simulink library "full_bridge_three_level_ttype_ideal_switch_based_model"  (R2025b)
settings: Solver=VariableStepAuto  StartTime=0.0  StopTime=10.0  RelTol=1e-3
libraries: nesl_utility x10, $bdroot x7, fl_lib x5
settings Model: Creator=dbagn  LastModifiedBy=dbagn

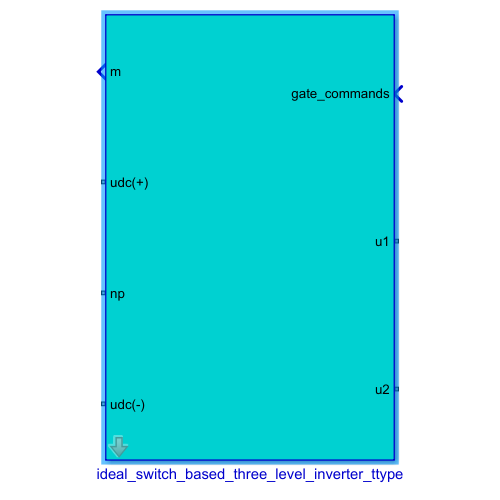
[thumbnail: Simulink's stored preview of the top-level diagram]
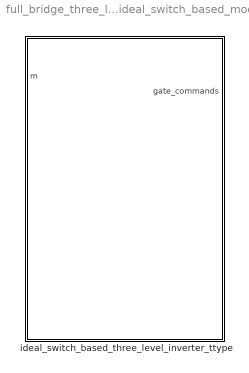
== system full_bridge_three_level_ttype_ideal_switch_based_model ==
  ideal_switch_based_three_level_inverter_ttype : Subsystem  mask{Vth=5.5, Ron=1.5e-3, Vdon_diode=2, Rdon_diode=0.15e-3, Csnubber=10e-9, Rsnubber=2200}

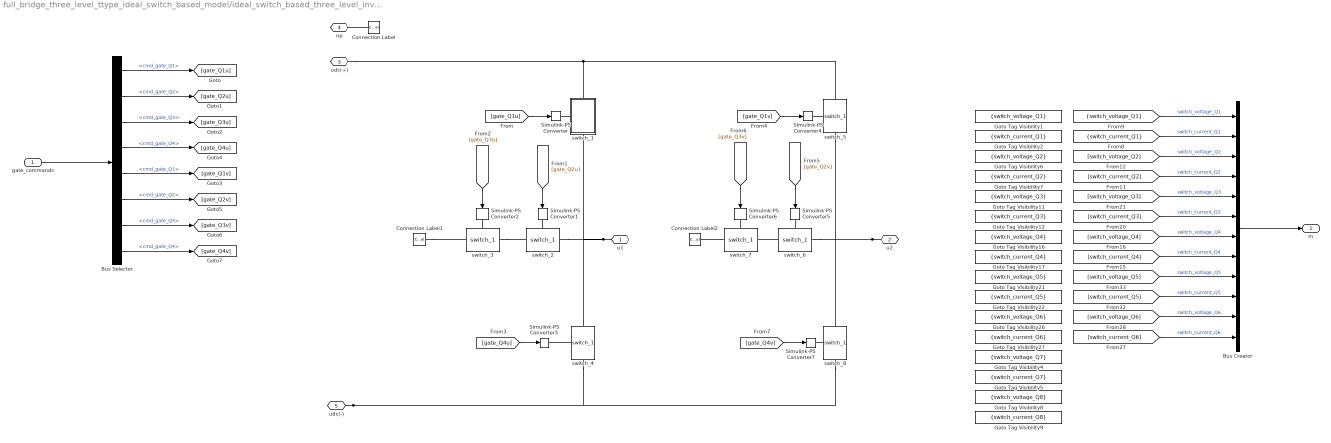
== system full_bridge_three_level_ttype_ideal_switch_based_model/ideal_switch_based_three_level_inverter_ttype ==
  gate_commands : Inport
  Bus Creator : BusCreator  Inputs=12
  Bus Selector : BusSelector  OutputSignals=gate_cmds_ph1.cmd_gate_Q1,gate_cmds_ph1.cmd_gate_Q2,gate_cmds_ph1.cmd_gate_Q3,gate_cmds_ph1.cmd_gate_Q4,gate_cmds_ph2.cmd_gate_Q1,gate_cmds_ph2.cmd_gate_Q2,gate_cmds_ph2.cmd_gate_Q3,gate_cmds_ph2.cmd_gate_Q4
  Connection Label : ConnectionLabel  Label=np
  Connection Label1 : ConnectionLabel  Label=np
  Connection Label2 : ConnectionLabel  Label=np
  Goto Tag Visibility1 : GotoTagVisibility  GotoTag=switch_voltage_Q1
  Goto Tag Visibility11 : GotoTagVisibility  GotoTag=switch_voltage_Q3
  Goto Tag Visibility12 : GotoTagVisibility  GotoTag=switch_current_Q3
  Goto Tag Visibility16 : GotoTagVisibility  GotoTag=switch_voltage_Q4
  Goto Tag Visibility17 : GotoTagVisibility  GotoTag=switch_current_Q4
  Goto Tag Visibility2 : GotoTagVisibility  GotoTag=switch_current_Q1
  Goto Tag Visibility21 : GotoTagVisibility  GotoTag=switch_voltage_Q5
  Goto Tag Visibility22 : GotoTagVisibility  GotoTag=switch_current_Q5
  Goto Tag Visibility26 : GotoTagVisibility  GotoTag=switch_voltage_Q6
  Goto Tag Visibility27 : GotoTagVisibility  GotoTag=switch_current_Q6
  Goto Tag Visibility4 : GotoTagVisibility  GotoTag=switch_voltage_Q7
  Goto Tag Visibility5 : GotoTagVisibility  GotoTag=switch_current_Q7
  Goto Tag Visibility6 : GotoTagVisibility  GotoTag=switch_voltage_Q2
  Goto Tag Visibility7 : GotoTagVisibility  GotoTag=switch_current_Q2
  Goto Tag Visibility8 : GotoTagVisibility  GotoTag=switch_voltage_Q8
  Goto Tag Visibility9 : GotoTagVisibility  GotoTag=switch_current_Q8
  Simulink-PS Converter{,1..7} (8 alike) : nesl_utility/Simulink-PS Converter  PhysicalDomain=network_engine_domain  SubClassName=ps_input  LeftPortType=input  RightPortType=output  PseudoPeriodic=off  Frequencies=[]  NoiseDistribution=none  NoiseParameters=[]  Unit=1  AffineConversion=on  FilteringAndDerivatives=provide  SimscapeFilterOrder=1  InputFilterTimeConstant=0.001  UdotUserProvided=0
  switch_1 : Subsystem
      settings: PortSchema="{\"entries\":[{\"content\":{\"sides\":[{\"content\":{\"connectorIds\":[\"LConn1\"]},\"type\":\"ConnectorPlacement.EquallySpacedRectSide\",\"uuid\":\"9277da8d-d460-43e6-8478-dd662f15d226\"},{\"content\":{\"connectorIds\":[],\"side\":\"RIGHT\"},\"type\":\"ConnectorPlacement.EquallySpacedRectSide\",\"uuid\":\"a7ece396-f1d9-4f4f-a05b-db1fc65d6e1d\"},{\"content\":{\"connectorIds\":[\"LConn2\"],\"side\":\"TOP\"},\"type\":\"ConnectorPlacement.EquallySpacedRectSide\",\"uuid\":\"fdd70777-e9cf-4317-afb6-cae87f75d5b0\"},{\"content\":{\"connectorIds\":[\"RConn1\"],\"side\":\"BOTTOM\"},\"type\":\"ConnectorPlacement.EquallySpacedRectSide\",\"uuid\":\"2353ed68-b1a1-4775-9ca9-31e268d5443b\"}]},\"type\":\"ConnectorPlacement.EquallySpacedConnector\",\"uuid\":\"d5479f4c-4e65-4791-adcb-73df11f88590\"}],\"packageUris\":[\"http://schema.mathworks.com/mf0/Connector/R2020b\"],\"version\":\"1.0\"}"
  switch_2 : $bdroot/ideal_switch_based_three_level_inverter_ttype/switch_1  SystemSampleTime=-1  VariantActivationTime=update diagram  EmptyChoice=off  PassThrough=off  PassThroughVariantControl=(default)  EmptyChoiceVariantControl=(default)  AllowFlexibleInterface=on  Latency=0  AutoFrameSizeCalculation=off
      link override Goto3: GotoTag=switch_voltage_Q2
      link override Goto6: GotoTag=switch_current_Q2
      settings: PortSchema="{\"entries\":[{\"content\":{\"sides\":[{\"content\":{\"connectorIds\":[\"LConn1\"]},\"type\":\"ConnectorPlacement.EquallySpacedRectSide\",\"uuid\":\"9277da8d-d460-43e6-8478-dd662f15d226\"},{\"content\":{\"connectorIds\":[],\"side\":\"RIGHT\"},\"type\":\"ConnectorPlacement.EquallySpacedRectSide\",\"uuid\":\"a7ece396-f1d9-4f4f-a05b-db1fc65d6e1d\"},{\"content\":{\"connectorIds\":[\"LConn2\"],\"side\":\"TOP\"},\"type\":\"ConnectorPlacement.EquallySpacedRectSide\",\"uuid\":\"fdd70777-e9cf-4317-afb6-cae87f75d5b0\"},{\"content\":{\"connectorIds\":[\"RConn1\"],\"side\":\"BOTTOM\"},\"type\":\"ConnectorPlacement.EquallySpacedRectSide\",\"uuid\":\"2353ed68-b1a1-4775-9ca9-31e268d5443b\"}]},\"type\":\"ConnectorPlacement.EquallySpacedConnector\",\"uuid\":\"d5479f4c-4e65-4791-adcb-73df11f88590\"}],\"packageUris\":[\"http://schema.mathworks.com/mf0/Connector/R2020b\"],\"version\":\"1.0\"}"
  switch_3 : $bdroot/ideal_switch_based_three_level_inverter_ttype/switch_1  SystemSampleTime=-1  VariantActivationTime=update diagram  EmptyChoice=off  PassThrough=off  PassThroughVariantControl=(default)  EmptyChoiceVariantControl=(default)  AllowFlexibleInterface=on  Latency=0  AutoFrameSizeCalculation=off
      link override Goto3: GotoTag=switch_voltage_Q3
      link override Goto6: GotoTag=switch_current_Q3
      settings: PortSchema="{\"entries\":[{\"content\":{\"sides\":[{\"content\":{\"connectorIds\":[\"LConn1\"]},\"type\":\"ConnectorPlacement.EquallySpacedRectSide\",\"uuid\":\"9277da8d-d460-43e6-8478-dd662f15d226\"},{\"content\":{\"connectorIds\":[],\"side\":\"RIGHT\"},\"type\":\"ConnectorPlacement.EquallySpacedRectSide\",\"uuid\":\"a7ece396-f1d9-4f4f-a05b-db1fc65d6e1d\"},{\"content\":{\"connectorIds\":[\"LConn2\"],\"side\":\"TOP\"},\"type\":\"ConnectorPlacement.EquallySpacedRectSide\",\"uuid\":\"fdd70777-e9cf-4317-afb6-cae87f75d5b0\"},{\"content\":{\"connectorIds\":[\"RConn1\"],\"side\":\"BOTTOM\"},\"type\":\"ConnectorPlacement.EquallySpacedRectSide\",\"uuid\":\"2353ed68-b1a1-4775-9ca9-31e268d5443b\"}]},\"type\":\"ConnectorPlacement.EquallySpacedConnector\",\"uuid\":\"d5479f4c-4e65-4791-adcb-73df11f88590\"}],\"packageUris\":[\"http://schema.mathworks.com/mf0/Connector/R2020b\"],\"version\":\"1.0\"}"
  switch_4 : $bdroot/ideal_switch_based_three_level_inverter_ttype/switch_1  SystemSampleTime=-1  VariantActivationTime=update diagram  EmptyChoice=off  PassThrough=off  PassThroughVariantControl=(default)  EmptyChoiceVariantControl=(default)  AllowFlexibleInterface=on  Latency=0  AutoFrameSizeCalculation=off
      link override Goto3: GotoTag=switch_voltage_Q4
      link override Goto6: GotoTag=switch_current_Q4
      settings: PortSchema="{\"entries\":[{\"content\":{\"sides\":[{\"content\":{\"connectorIds\":[\"LConn1\"]},\"type\":\"ConnectorPlacement.EquallySpacedRectSide\",\"uuid\":\"9277da8d-d460-43e6-8478-dd662f15d226\"},{\"content\":{\"connectorIds\":[],\"side\":\"RIGHT\"},\"type\":\"ConnectorPlacement.EquallySpacedRectSide\",\"uuid\":\"a7ece396-f1d9-4f4f-a05b-db1fc65d6e1d\"},{\"content\":{\"connectorIds\":[\"LConn2\"],\"side\":\"TOP\"},\"type\":\"ConnectorPlacement.EquallySpacedRectSide\",\"uuid\":\"fdd70777-e9cf-4317-afb6-cae87f75d5b0\"},{\"content\":{\"connectorIds\":[\"RConn1\"],\"side\":\"BOTTOM\"},\"type\":\"ConnectorPlacement.EquallySpacedRectSide\",\"uuid\":\"2353ed68-b1a1-4775-9ca9-31e268d5443b\"}]},\"type\":\"ConnectorPlacement.EquallySpacedConnector\",\"uuid\":\"d5479f4c-4e65-4791-adcb-73df11f88590\"}],\"packageUris\":[\"http://schema.mathworks.com/mf0/Connector/R2020b\"],\"version\":\"1.0\"}"
  switch_5 : $bdroot/ideal_switch_based_three_level_inverter_ttype/switch_1  SystemSampleTime=-1  VariantActivationTime=update diagram  EmptyChoice=off  PassThrough=off  PassThroughVariantControl=(default)  EmptyChoiceVariantControl=(default)  AllowFlexibleInterface=on  Latency=0  AutoFrameSizeCalculation=off
      link override Goto3: GotoTag=switch_voltage_Q5
      link override Goto6: GotoTag=switch_current_Q5
      settings: PortSchema="{\"entries\":[{\"content\":{\"sides\":[{\"content\":{\"connectorIds\":[\"LConn1\"]},\"type\":\"ConnectorPlacement.EquallySpacedRectSide\",\"uuid\":\"9277da8d-d460-43e6-8478-dd662f15d226\"},{\"content\":{\"connectorIds\":[],\"side\":\"RIGHT\"},\"type\":\"ConnectorPlacement.EquallySpacedRectSide\",\"uuid\":\"a7ece396-f1d9-4f4f-a05b-db1fc65d6e1d\"},{\"content\":{\"connectorIds\":[\"LConn2\"],\"side\":\"TOP\"},\"type\":\"ConnectorPlacement.EquallySpacedRectSide\",\"uuid\":\"fdd70777-e9cf-4317-afb6-cae87f75d5b0\"},{\"content\":{\"connectorIds\":[\"RConn1\"],\"side\":\"BOTTOM\"},\"type\":\"ConnectorPlacement.EquallySpacedRectSide\",\"uuid\":\"2353ed68-b1a1-4775-9ca9-31e268d5443b\"}]},\"type\":\"ConnectorPlacement.EquallySpacedConnector\",\"uuid\":\"d5479f4c-4e65-4791-adcb-73df11f88590\"}],\"packageUris\":[\"http://schema.mathworks.com/mf0/Connector/R2020b\"],\"version\":\"1.0\"}"
  switch_6 : $bdroot/ideal_switch_based_three_level_inverter_ttype/switch_1  SystemSampleTime=-1  VariantActivationTime=update diagram  EmptyChoice=off  PassThrough=off  PassThroughVariantControl=(default)  EmptyChoiceVariantControl=(default)  AllowFlexibleInterface=on  Latency=0  AutoFrameSizeCalculation=off
      link override Goto3: GotoTag=switch_voltage_Q6
      link override Goto6: GotoTag=switch_current_Q6
      settings: PortSchema="{\"entries\":[{\"content\":{\"sides\":[{\"content\":{\"connectorIds\":[\"LConn1\"]},\"type\":\"ConnectorPlacement.EquallySpacedRectSide\",\"uuid\":\"9277da8d-d460-43e6-8478-dd662f15d226\"},{\"content\":{\"connectorIds\":[],\"side\":\"RIGHT\"},\"type\":\"ConnectorPlacement.EquallySpacedRectSide\",\"uuid\":\"a7ece396-f1d9-4f4f-a05b-db1fc65d6e1d\"},{\"content\":{\"connectorIds\":[\"LConn2\"],\"side\":\"TOP\"},\"type\":\"ConnectorPlacement.EquallySpacedRectSide\",\"uuid\":\"fdd70777-e9cf-4317-afb6-cae87f75d5b0\"},{\"content\":{\"connectorIds\":[\"RConn1\"],\"side\":\"BOTTOM\"},\"type\":\"ConnectorPlacement.EquallySpacedRectSide\",\"uuid\":\"2353ed68-b1a1-4775-9ca9-31e268d5443b\"}]},\"type\":\"ConnectorPlacement.EquallySpacedConnector\",\"uuid\":\"d5479f4c-4e65-4791-adcb-73df11f88590\"}],\"packageUris\":[\"http://schema.mathworks.com/mf0/Connector/R2020b\"],\"version\":\"1.0\"}"
  switch_7 : $bdroot/ideal_switch_based_three_level_inverter_ttype/switch_1  SystemSampleTime=-1  VariantActivationTime=update diagram  EmptyChoice=off  PassThrough=off  PassThroughVariantControl=(default)  EmptyChoiceVariantControl=(default)  AllowFlexibleInterface=on  Latency=0  AutoFrameSizeCalculation=off
      link override Goto3: GotoTag=switch_voltage_Q7
      link override Goto6: GotoTag=switch_current_Q7
      settings: PortSchema="{\"entries\":[{\"content\":{\"sides\":[{\"content\":{\"connectorIds\":[\"LConn1\"]},\"type\":\"ConnectorPlacement.EquallySpacedRectSide\",\"uuid\":\"9277da8d-d460-43e6-8478-dd662f15d226\"},{\"content\":{\"connectorIds\":[],\"side\":\"RIGHT\"},\"type\":\"ConnectorPlacement.EquallySpacedRectSide\",\"uuid\":\"a7ece396-f1d9-4f4f-a05b-db1fc65d6e1d\"},{\"content\":{\"connectorIds\":[\"LConn2\"],\"side\":\"TOP\"},\"type\":\"ConnectorPlacement.EquallySpacedRectSide\",\"uuid\":\"fdd70777-e9cf-4317-afb6-cae87f75d5b0\"},{\"content\":{\"connectorIds\":[\"RConn1\"],\"side\":\"BOTTOM\"},\"type\":\"ConnectorPlacement.EquallySpacedRectSide\",\"uuid\":\"2353ed68-b1a1-4775-9ca9-31e268d5443b\"}]},\"type\":\"ConnectorPlacement.EquallySpacedConnector\",\"uuid\":\"d5479f4c-4e65-4791-adcb-73df11f88590\"}],\"packageUris\":[\"http://schema.mathworks.com/mf0/Connector/R2020b\"],\"version\":\"1.0\"}"
  switch_8 : $bdroot/ideal_switch_based_three_level_inverter_ttype/switch_1  SystemSampleTime=-1  VariantActivationTime=update diagram  EmptyChoice=off  PassThrough=off  PassThroughVariantControl=(default)  EmptyChoiceVariantControl=(default)  AllowFlexibleInterface=on  Latency=0  AutoFrameSizeCalculation=off
      link override Goto3: GotoTag=switch_voltage_Q8
      link override Goto6: GotoTag=switch_current_Q8
      settings: PortSchema="{\"entries\":[{\"content\":{\"sides\":[{\"content\":{\"connectorIds\":[\"LConn1\"]},\"type\":\"ConnectorPlacement.EquallySpacedRectSide\",\"uuid\":\"9277da8d-d460-43e6-8478-dd662f15d226\"},{\"content\":{\"connectorIds\":[],\"side\":\"RIGHT\"},\"type\":\"ConnectorPlacement.EquallySpacedRectSide\",\"uuid\":\"a7ece396-f1d9-4f4f-a05b-db1fc65d6e1d\"},{\"content\":{\"connectorIds\":[\"LConn2\"],\"side\":\"TOP\"},\"type\":\"ConnectorPlacement.EquallySpacedRectSide\",\"uuid\":\"fdd70777-e9cf-4317-afb6-cae87f75d5b0\"},{\"content\":{\"connectorIds\":[\"RConn1\"],\"side\":\"BOTTOM\"},\"type\":\"ConnectorPlacement.EquallySpacedRectSide\",\"uuid\":\"2353ed68-b1a1-4775-9ca9-31e268d5443b\"}]},\"type\":\"ConnectorPlacement.EquallySpacedConnector\",\"uuid\":\"d5479f4c-4e65-4791-adcb-73df11f88590\"}],\"packageUris\":[\"http://schema.mathworks.com/mf0/Connector/R2020b\"],\"version\":\"1.0\"}"
  u1 : PMIOPort  Side=Left
  u2 : PMIOPort  Port=2  Side=Left
  udc(+) : PMIOPort  Port=3  Side=Right
  np : PMIOPort  Port=4  Side=Right
  udc(-) : PMIOPort  Port=5  Side=Right
  m : Outport
  wires:
  [gate_Q4u] -> Simulink-PS Converter3/1
  [gate_Q3u] -> Simulink-PS Converter2/1
  [gate_Q2u] -> Simulink-PS Converter1/1
  [gate_Q1u] -> Simulink-PS Converter/1
  [gate_Q1v] -> Simulink-PS Converter4/1
  [gate_Q2v] -> Simulink-PS Converter5/1
  [gate_Q3v] -> Simulink-PS Converter6/1
  [gate_Q4v] -> Simulink-PS Converter7/1
  gate_commands/1 -> Bus Selector/1
  Bus Selector/1 -> [gate_Q1u]  "<cmd_gate_Q1>"
  Bus Selector/3 -> [gate_Q3u]  "<cmd_gate_Q3>"
  Bus Selector/2 -> [gate_Q2u]  "<cmd_gate_Q2>"
  Bus Selector/4 -> [gate_Q4u]  "<cmd_gate_Q4>"
  Bus Selector/5 -> [gate_Q1v]  "<cmd_gate_Q1>"
  Bus Selector/6 -> [gate_Q2v]  "<cmd_gate_Q2>"
  Bus Selector/7 -> [gate_Q3v]  "<cmd_gate_Q3>"
  Bus Selector/8 -> [gate_Q4v]  "<cmd_gate_Q4>"
  [switch_current_Q4] -> Bus Creator/8  "switch_current_Q4"
  [switch_voltage_Q2] -> Bus Creator/3  "switch_voltage_Q2"
  [switch_voltage_Q3] -> Bus Creator/5  "switch_voltage_Q3"
  Bus Creator/1 -> m/1
  [switch_voltage_Q1] -> Bus Creator/1  "switch_voltage_Q1"
  [switch_current_Q6] -> Bus Creator/12  "switch_current_Q6"
  [switch_current_Q2] -> Bus Creator/4  "switch_current_Q2"
  [switch_current_Q3] -> Bus Creator/6  "switch_current_Q3"
  [switch_voltage_Q5] -> Bus Creator/9  "switch_voltage_Q5"
  [switch_voltage_Q4] -> Bus Creator/7  "switch_voltage_Q4"
  [switch_voltage_Q6] -> Bus Creator/11  "switch_voltage_Q6"
  [switch_current_Q1] -> Bus Creator/2  "switch_current_Q1"
  [switch_current_Q5] -> Bus Creator/10  "switch_current_Q5"
  connections:
  udc(+)/RConn1 -- switch_5/LConn2 -- switch_1/LConn2
  switch_4/LConn1 -- Simulink-PS Converter3/RConn1
  switch_3/LConn1 -- Simulink-PS Converter2/RConn1
  switch_2/LConn1 -- Simulink-PS Converter1/RConn1
  switch_1/LConn1 -- Simulink-PS Converter/RConn1
  switch_6/LConn1 -- Simulink-PS Converter5/RConn1
  switch_5/LConn1 -- Simulink-PS Converter4/RConn1
  switch_7/LConn1 -- Simulink-PS Converter6/RConn1
  switch_8/LConn1 -- Simulink-PS Converter7/RConn1
  Connection Label/LConn1 -- np/RConn1
  u1/RConn1 -- switch_2/RConn1 -- switch_4/LConn2 -- switch_1/RConn1
  udc(-)/RConn1 -- switch_8/RConn1 -- switch_4/RConn1
  u2/RConn1 -- switch_6/RConn1 -- switch_8/LConn2 -- switch_5/RConn1
  switch_3/LConn2 -- switch_2/LConn2
  Connection Label1/LConn1 -- switch_3/RConn1
  switch_7/RConn1 -- Connection Label2/LConn1
  switch_6/LConn2 -- switch_7/LConn2

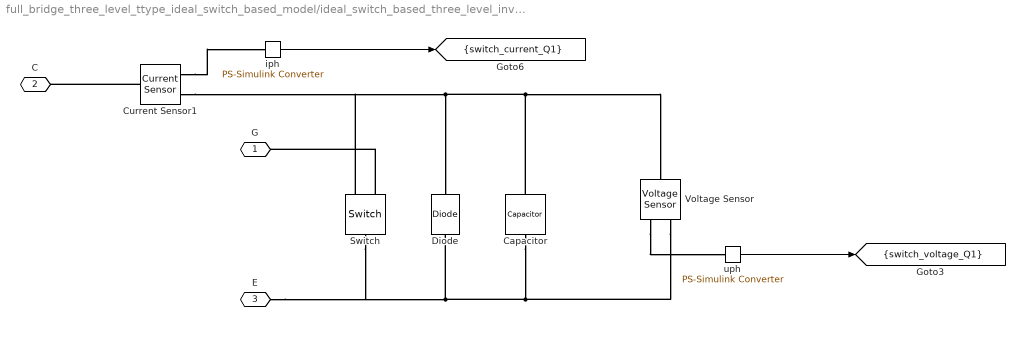
== system full_bridge_three_level_ttype_ideal_switch_based_model/ideal_switch_based_three_level_inverter_ttype/switch_1 ==
  Capacitor : fl_lib/Electrical/Electrical Elements/Capacitor  c=Csnubber F  r=Rsnubber Ohm  g=0 1/Ohm  i_specify=off  i_priority=None  i=0 A  i_nominal_specify=off  i_nominal_value=1  i_nominal_unit=A  v_specify=off  v_priority=None  v=0 V  v_nominal_specify=off  v_nominal_value=1  v_nominal_unit=V  vc_specify=off  vc_priority=High  vc=0 V  vc_nominal_specify=off  vc_nominal_value=1  vc_nominal_unit=V
  Current Sensor1 : fl_lib/Electrical/Electrical Sensors/Current Sensor
  Diode : fl_lib/Electrical/Electrical Elements/Diode  Vf=Vdon_diode V  Ron=Rdon_diode Ohm  Goff=1e-8 1/Ohm  i_specify=off  i_priority=None  i=0 A  i_nominal_specify=off  i_nominal_value=1  i_nominal_unit=A  v_specify=off  v_priority=None  v=0 V  v_nominal_specify=off  v_nominal_value=1  v_nominal_unit=V
  Switch : fl_lib/Electrical/Electrical Elements/Switch  R_closed=Ron Ohm  G_open=1e-8 1/Ohm  Threshold=Vth  i_specify=off  i_priority=None  i=0 A  i_nominal_specify=off  i_nominal_value=1  i_nominal_unit=A  v_specify=off  v_priority=None  v=0 V  v_nominal_specify=off  v_nominal_value=1  v_nominal_unit=V
  Voltage Sensor : fl_lib/Electrical/Electrical Sensors/Voltage Sensor
  iph : nesl_utility/PS-Simulink Converter  PhysicalDomain=network_engine_domain  SubClassName=ps_output  LeftPortType=input  RightPortType=output  PseudoPeriodic=off  Frequencies=[]  VectorFormat=1-D array  Unit=A  AffineConversion=off
  uph : nesl_utility/PS-Simulink Converter  PhysicalDomain=network_engine_domain  SubClassName=ps_output  LeftPortType=input  RightPortType=output  PseudoPeriodic=off  Frequencies=[]  VectorFormat=1-D array  Unit=V  AffineConversion=off
  G : PMIOPort  Side=Left
  C : PMIOPort  Port=2  Side=Left
  E : PMIOPort  Port=3  Side=Right
  tag scope: switch_current_Q1=scoped, switch_voltage_Q1=scoped
  wires:
  uph/1 -> [switch_voltage_Q1]
  iph/1 -> [switch_current_Q1]
  connections:
  Capacitor/RConn1 -- Voltage Sensor/RConn2 -- E/RConn1 -- Switch/LConn1 -- Diode/LConn1
  Switch/RConn1 -- G/RConn1
  Capacitor/LConn1 -- Voltage Sensor/LConn1 -- Switch/RConn2 -- Current Sensor1/RConn2 -- Diode/RConn1
  Current Sensor1/RConn1 -- iph/LConn1
  Voltage Sensor/RConn1 -- uph/LConn1
  Current Sensor1/LConn1 -- C/RConn1
